simulink model "IntakeManifold"  (R2025b)
settings: Solver=ode1  StartTime=0.0  StopTime=10.0  FixedStep=0.001  RelTol=1e-3
undefined symbols (not defined in the file): pm0, R, Vm
settings Model: Creator=williamvandevoir  LastModifiedBy=williamvandevoir

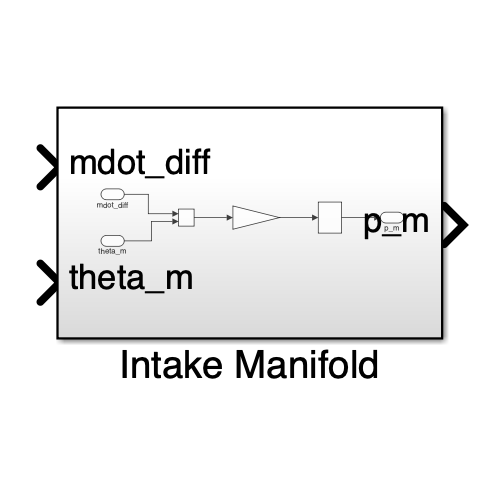
[thumbnail: Simulink's stored preview of the top-level diagram]
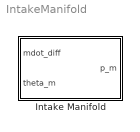
== system IntakeManifold ==
  Intake Manifold : Subsystem  Description=Adapted from Intake Manifold Exercise (pressure dynamics only): dp_m/dt = R*theta_m/Vm*(mdot_alpha - mdot_beta). One state; theta_m is an input; R instead of kappa*R.

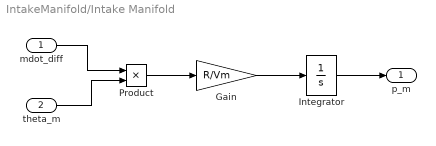
== system IntakeManifold/Intake Manifold ==
  mdot_diff : Inport
  theta_m : Inport  Port=2
  Gain : Gain  Gain=R/Vm
  Integrator : Integrator  InitialCondition=pm0
  Product : Product
  p_m : Outport
  wires:
  mdot_diff/1 -> Product/1
  theta_m/1 -> Product/2
  Product/1 -> Gain/1
  Gain/1 -> Integrator/1
  Integrator/1 -> p_m/1
